simulink model "elp_lv_demand"  (R2026b)
settings: Solver=VariableStepAuto
undefined symbols (not defined in the file or in its folder): P, Ts
settings Model: Creator=aomar  LastModifiedBy=aomar

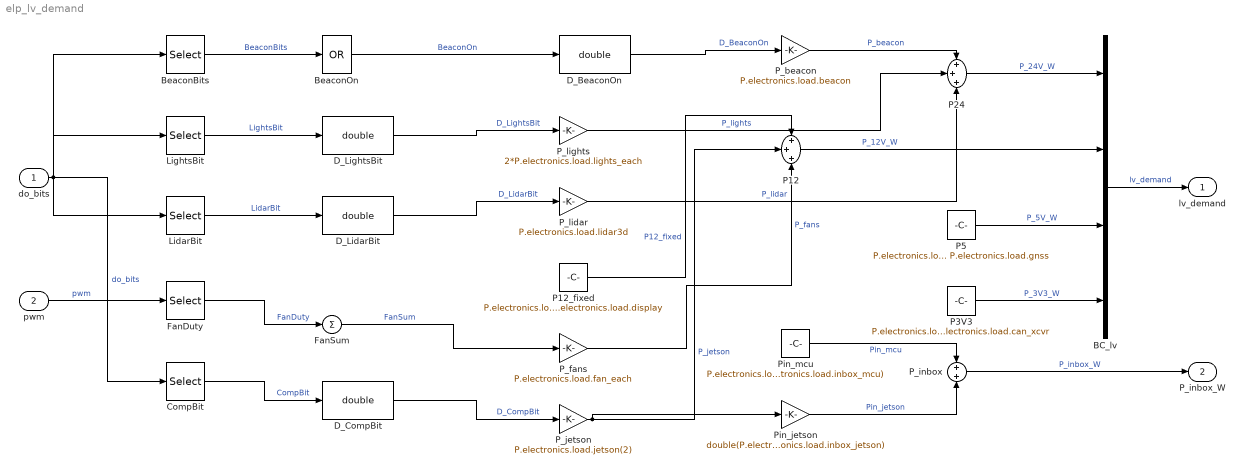
== system elp_lv_demand ==
  do_bits : Inport  OutDataTypeStr=boolean  PortDimensions=32  SampleTime=Ts.ctrl
  pwm : Inport  Port=2  OutDataTypeStr=double  PortDimensions=4  SampleTime=Ts.ctrl
  BC_lv : BusCreator  Inputs=4  OutDataTypeStr=Bus: Bus_LV_LoadDemand  NonVirtualBus=on
      settings: InheritFromInputs=off
  BeaconBits : Selector  InputPortWidth=32  IndexOptions=Index vector (dialog)  Indices=[1 + P.electronics.do.beacon_green, 1 + P.electronics.do.beacon_amber, 1 + P.electronics.do.beacon_red, 1 + P.electronics.do.buzzer]  OutputSizes=1
  BeaconOn : Logic  Operator=OR  Inputs=1  AllPortsSameDT=off  OutDataTypeStr=boolean
  CompBit : Selector  InputPortWidth=32  IndexOptions=Index vector (dialog)  Indices=1 + P.electronics.do.companion_pwr_en  OutputSizes=1
  D_BeaconOn : DataTypeConversion  OutDataTypeStr=double  RndMeth=Nearest
  D_CompBit : DataTypeConversion  OutDataTypeStr=double  RndMeth=Nearest
  D_LidarBit : DataTypeConversion  OutDataTypeStr=double  RndMeth=Nearest
  D_LightsBit : DataTypeConversion  OutDataTypeStr=double  RndMeth=Nearest
  FanDuty : Selector  InputPortWidth=4  IndexOptions=Index vector (dialog)  Indices=[3 4]  OutputSizes=1
  FanSum : Sum  Inputs=+
  LidarBit : Selector  InputPortWidth=32  IndexOptions=Index vector (dialog)  Indices=1 + P.electronics.do.lidar_pwr_en  OutputSizes=1
  LightsBit : Selector  InputPortWidth=32  IndexOptions=Index vector (dialog)  Indices=1 + P.electronics.do.work_lights  OutputSizes=1
  P12 : Sum  Inputs=+++
  P12_fixed : Constant  Value=P.electronics.load.mcu + P.electronics.load.modem + P.electronics.load.cams + P.electronics.load.display  OutDataTypeStr=double  SampleTime=Ts.ctrl
  P24 : Sum  Inputs=+++
  P3V3 : Constant  Value=P.electronics.load.imu + P.electronics.load.can_xcvr  OutDataTypeStr=double  SampleTime=Ts.ctrl
  P5 : Constant  Value=P.electronics.load.rc_rx + P.electronics.load.gnss  OutDataTypeStr=double  SampleTime=Ts.ctrl
  P_beacon : Gain  Gain=P.electronics.load.beacon
  P_fans : Gain  Gain=P.electronics.load.fan_each
  P_inbox : Sum
  P_jetson : Gain  Gain=P.electronics.load.jetson(2)
  P_lidar : Gain  Gain=P.electronics.load.lidar3d
  P_lights : Gain  Gain=2*P.electronics.load.lights_each
  Pin_jetson : Gain  Gain=double(P.electronics.load.inbox_jetson)
  Pin_mcu : Constant  Value=P.electronics.load.mcu*double(P.electronics.load.inbox_mcu)  OutDataTypeStr=double  SampleTime=Ts.ctrl
  lv_demand : Outport  OutDataTypeStr=Bus: Bus_LV_LoadDemand
  P_inbox_W : Outport  Port=2  OutDataTypeStr=double
  wires:
  do_bits/1 -> CompBit/1, BeaconBits/1, LightsBit/1, LidarBit/1  "do_bits"
  pwm/1 -> FanDuty/1  "pwm"
  BeaconBits/1 -> BeaconOn/1  "BeaconBits"
  LightsBit/1 -> D_LightsBit/1  "LightsBit"
  LidarBit/1 -> D_LidarBit/1  "LidarBit"
  FanDuty/1 -> FanSum/1  "FanDuty"
  CompBit/1 -> D_CompBit/1  "CompBit"
  FanSum/1 -> P_fans/1  "FanSum"
  BeaconOn/1 -> D_BeaconOn/1  "BeaconOn"
  D_LightsBit/1 -> P_lights/1  "D_LightsBit"
  D_LidarBit/1 -> P_lidar/1  "D_LidarBit"
  D_CompBit/1 -> P_jetson/1  "D_CompBit"
  P_lights/1 -> P24/2  "P_lights"
  P_lidar/1 -> P24/3  "P_lidar"
  P12_fixed/1 -> P12/1  "P12_fixed"
  P_fans/1 -> P12/3  "P_fans"
  P_jetson/1 -> P12/2, Pin_jetson/1  "P_jetson"
  D_BeaconOn/1 -> P_beacon/1  "D_BeaconOn"
  P12/1 -> BC_lv/2  "P_12V_W"
  P_beacon/1 -> P24/1  "P_beacon"
  Pin_mcu/1 -> P_inbox/1  "Pin_mcu"
  Pin_jetson/1 -> P_inbox/2  "Pin_jetson"
  P24/1 -> BC_lv/1  "P_24V_W"
  P_inbox/1 -> P_inbox_W/1  "P_inbox_W"
  P5/1 -> BC_lv/3  "P_5V_W"
  P3V3/1 -> BC_lv/4  "P_3V3_W"
  BC_lv/1 -> lv_demand/1  "lv_demand"
